simulink model "PvarrayParrallel"  (R2025a)
settings: Solver=ode23tb  StartTime=0.0  StopTime=0.2  RelTol=1e-3
libraries: spsDiodeLib x7, spsPVArrayLib x6, spsSeriesRLCBranchLib x6, slpidlib x2, spsPower3phPhasorLib x2, spsThreePhaseVIMeasurementLib x2, spsVoltageMeasurementLib x2, spsCurrentMeasurementLib x1, spsIGBTDiodeLib x1, eeGeneralControl x1, spsPLL3phLib x1, spsPWMGenerator2LevelLib x1
settings Model: Creator=BIT  LastModifiedBy=BIT

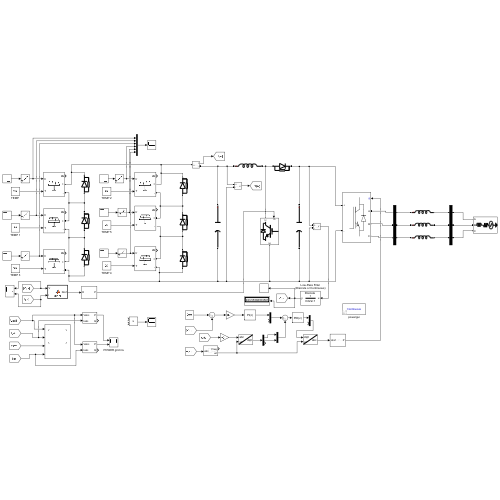
[thumbnail: Simulink's stored preview of the top-level diagram]
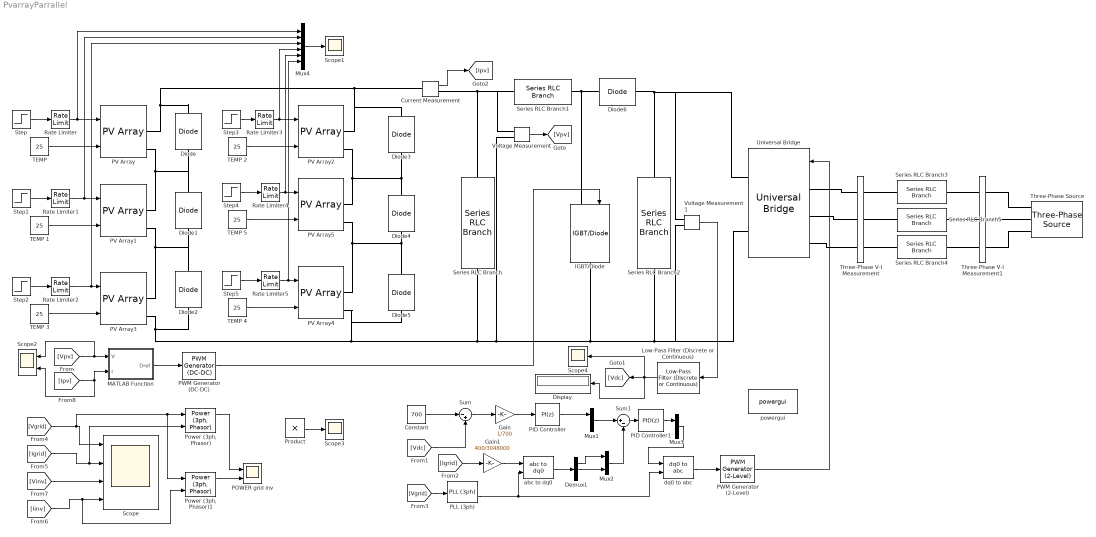
== system PvarrayParrallel ==
  Constant : Constant  Value=700
  Current Measurement : spsCurrentMeasurementLib/Current Measurement  PhasorSimulation=off  OutputType=Complex  PSBequivalent=0
  Demux1 : Demux  Outputs=3
  Diode{,1..6} (7 alike) : spsDiodeLib/Diode  Ron=0.001  Lon=0  Vf=0.8  IC=0  UseSnubber=0  Rs=500  Cs=250e-9  Measurements=off
  Display : Display
  Gain : Gain  Gain=1/700
  Gain1 : Gain  Gain=400/3048000
  IGBT/Diode : spsIGBTDiodeLib/IGBT//Diode  Ron=1e-3  Rs=1e5  Cs=inf  Measurements=off
  Low-Pass Filter (Discrete or Continuous) : eeGeneralControl/Low-Pass Filter (Discrete or Continuous)  K=1  T=1/50  B=inf  A=-inf  init_option=Inherited from block input  x0=0  Ts=1e-06
  MATLAB Function : MATLAB Function  TreatAsAtomicUnit=on
  Mux1 : Mux  Inputs=2
  Mux2 : Mux  Inputs=2
  Mux3 : Mux  Inputs=2
  Mux4 : Mux  Inputs=6
  PID Controller : slpidlib/PID Controller  Controller=PI  Form=Parallel  TimeDomain=Discrete-time  UseExternalTs=off  SampleTime=-1  IntegratorMethod=Forward Euler  FilterMethod=Forward Euler  ControllerParametersSource=internal  P=100  I=100  UseKiTs=off  D=0  UseExternalDerivativeSource=off  N=100  UseFilter=on  TunerSelectOption=Transfer Function Based (PID Tuner App)  InitialConditionSource=internal  InitialConditionForIntegrator=0  InitialConditionForFilter=0  DifferentiatorICPrevScaledInput=0  ExternalReset=none  TrackingMode=off  Kt=1  LimitOutput=off  SatLimitsSource=internal  UpperSaturationLimit=inf  LowerSaturationLimit=-inf  LinearizeAsGain=on  AntiWindupMode=none  Kb=1  LimitIntegrator=off  UpperIntegratorSaturationLimit=inf  LowerIntegratorSaturationLimit=-inf  POutMin=[]  POutMax=[]  IOutMin=[]  IOutMax=[]  DOutMin=[]  DOutMax=[]  NOutMin=[]  NOutMax=[]  SumOutMin=[]  SumOutMax=[]  SaturationOutMin=[]  SaturationOutMax=[]  PParamMin=[]  PParamMax=[]  IParamMin=[]  IParamMax=[]  DParamMin=[]  DParamMax=[]  NParamMin=[]  NParamMax=[]  KbParamMin=[]  KbParamMax=[]  KtParamMin=[]  KtParamMax=[]  KbOutMin=[]  KbOutMax=[]  KtOutMin=[]  KtOutMax=[]  IntegratorOutMin=[]  IntegratorOutMax=[]  FilterOutMin=[]  FilterOutMax=[]  SumI1OutMin=[]  SumI1OutMax=[]  SumI2OutMin=[]  SumI2OutMax=[]  SumI3OutMin=[]  SumI3OutMax=[]  SumI4OutMin=[]  SumI4OutMax=[]  SumDOutMin=[]  SumDOutMax=[]  DifferentiatorOutMin=[]  DifferentiatorOutMax=[]  FilterDiffOutCoefMin=[]  FilterDiffOutCoefMax=[]  ReciprocalOutMin=[]  ReciprocalOutMax=[]  SumDenOutMin=[]  SumDenOutMax=[]  SumNumOutMin=[]  SumNumOutMax=[]  DivideOutMin=[]  DivideOutMax=[]  UdiffTsProdOutMin=[]  UdiffTsProdOutMax=[]  NTsProdOutMin=[]  NTsProdOutMax=[]  UintegralTsProdOutMin=[]  UintegralTsProdOutMax=[]  UngainTsProdOutMin=[]  UngainTsProdOutMax=[]  ClampingZeroOutDataTypeStr=Inherit: Inherit via back propagation  ClampingZeroOutMin=[]  ClampingZeroOutMax=[]  FilterDenConstantOutDataTypeStr=Inherit: Inherit via back propagation  FilterDenConstantOutMin=[]  FilterDenConstantOutMax=[]  PCopyOutDataTypeStr=Inherit: Inherit via back propagation  PCopyOutMin=[]  PCopyOutMax=[]  NCopyOutDataTypeStr=Inherit: Inherit via back propagation  NCopyOutMin=[]  NCopyOutMax=[]  IntegratorContinuousStateAttributes=''  IntegratorStateMustResolveToSignalObject=off  IntegratorRTWStateStorageClass=Auto  FilterContinuousStateAttributes=''  FilterStateMustResolveToSignalObject=off  FilterRTWStateStorageClass=Auto  ParallelPVariant=InternalParameters  IdealPVariant=Disabled  IVariant=InternalParameters  DVariant=Disabled  IntegratorVariant=Discrete  SatVariant=Disabled  AWVariant=Passthrough  PCopyVariant=Disabled  TRVariant=Disabled  FdbkBlocksVariant=Forward  IdealPFdbkVariant=Disabled  SatFdbkVariant=Disabled  DerivativeFilterVariant=Disabled  NVariant=Disabled  NCopyVariant=Disabled_SignalSpec  FilterICVariant=Disabled  IntegratorICVariant=InternalICs  ExternalResetVariant=Disabled  TRSumVariant=Passthrough  SumFdbkVariant=Disabled  SumVariant=Sum_PI  TsampFilterVariant=InternalTs  TsampNgainVariant=Passthrough  TsampIntegralVariant=Disabled_SignalSpec  ExternalSaturationOutDataTypeStr=Inherit: Same as second input  DerivativeSourceVariant=Disabled  PreIntVariant=InternalPreInt
  PID Controller1 : slpidlib/PID Controller  Controller=PID  Form=Parallel  TimeDomain=Discrete-time  UseExternalTs=off  SampleTime=-1  IntegratorMethod=Forward Euler  FilterMethod=Forward Euler  ControllerParametersSource=internal  P=1  I=1  UseKiTs=off  D=0  UseExternalDerivativeSource=off  N=100  UseFilter=on  TunerSelectOption=Transfer Function Based (PID Tuner App)  InitialConditionSource=internal  InitialConditionForIntegrator=0  InitialConditionForFilter=0  DifferentiatorICPrevScaledInput=0  ExternalReset=none  TrackingMode=off  Kt=1  LimitOutput=off  SatLimitsSource=internal  UpperSaturationLimit=inf  LowerSaturationLimit=-inf  LinearizeAsGain=on  AntiWindupMode=none  Kb=1  LimitIntegrator=off  UpperIntegratorSaturationLimit=inf  LowerIntegratorSaturationLimit=-inf  POutMin=[]  POutMax=[]  IOutMin=[]  IOutMax=[]  DOutMin=[]  DOutMax=[]  NOutMin=[]  NOutMax=[]  SumOutMin=[]  SumOutMax=[]  SaturationOutMin=[]  SaturationOutMax=[]  PParamMin=[]  PParamMax=[]  IParamMin=[]  IParamMax=[]  DParamMin=[]  DParamMax=[]  NParamMin=[]  NParamMax=[]  KbParamMin=[]  KbParamMax=[]  KtParamMin=[]  KtParamMax=[]  KbOutMin=[]  KbOutMax=[]  KtOutMin=[]  KtOutMax=[]  IntegratorOutMin=[]  IntegratorOutMax=[]  FilterOutMin=[]  FilterOutMax=[]  SumI1OutMin=[]  SumI1OutMax=[]  SumI2OutMin=[]  SumI2OutMax=[]  SumI3OutMin=[]  SumI3OutMax=[]  SumI4OutMin=[]  SumI4OutMax=[]  SumDOutMin=[]  SumDOutMax=[]  DifferentiatorOutMin=[]  DifferentiatorOutMax=[]  FilterDiffOutCoefMin=[]  FilterDiffOutCoefMax=[]  ReciprocalOutMin=[]  ReciprocalOutMax=[]  SumDenOutMin=[]  SumDenOutMax=[]  SumNumOutMin=[]  SumNumOutMax=[]  DivideOutMin=[]  DivideOutMax=[]  UdiffTsProdOutMin=[]  UdiffTsProdOutMax=[]  NTsProdOutMin=[]  NTsProdOutMax=[]  UintegralTsProdOutMin=[]  UintegralTsProdOutMax=[]  UngainTsProdOutMin=[]  UngainTsProdOutMax=[]  ClampingZeroOutDataTypeStr=Inherit: Inherit via back propagation  ClampingZeroOutMin=[]  ClampingZeroOutMax=[]  FilterDenConstantOutDataTypeStr=Inherit: Inherit via back propagation  FilterDenConstantOutMin=[]  FilterDenConstantOutMax=[]  PCopyOutDataTypeStr=Inherit: Inherit via back propagation  PCopyOutMin=[]  PCopyOutMax=[]  NCopyOutDataTypeStr=Inherit: Inherit via back propagation  NCopyOutMin=[]  NCopyOutMax=[]  IntegratorContinuousStateAttributes=''  IntegratorStateMustResolveToSignalObject=off  IntegratorRTWStateStorageClass=Auto  FilterContinuousStateAttributes=''  FilterStateMustResolveToSignalObject=off  FilterRTWStateStorageClass=Auto  ParallelPVariant=InternalParameters  IdealPVariant=Disabled  IVariant=InternalParameters  DVariant=InternalParameters  IntegratorVariant=Discrete  SatVariant=Disabled  AWVariant=Passthrough  PCopyVariant=Disabled  TRVariant=Disabled  FdbkBlocksVariant=Forward  IdealPFdbkVariant=Disabled  SatFdbkVariant=Disabled  DerivativeFilterVariant=ForwardEulerFilter  NVariant=InternalParameters  NCopyVariant=Disabled  FilterICVariant=InternalICsFilter  IntegratorICVariant=InternalICs  ExternalResetVariant=Disabled  TRSumVariant=Passthrough  SumFdbkVariant=Disabled  SumVariant=Sum_PID  TsampFilterVariant=InternalTs  TsampNgainVariant=Passthrough  TsampIntegralVariant=Disabled_SignalSpec  ExternalSaturationOutDataTypeStr=Inherit: Same as second input  DerivativeSourceVariant=ErrorSignal  PreIntVariant=InternalPreInt
  PLL (3ph) : spsPLL3phLib/PLL (3ph)  Fmin=45  Par_Init=[0, 50]  ParK=[180, 3200, 1]  TcD=1e-4  MaxRateChangeFreq=12  FilterCutOffFreq=25  Ts=0  AGC=on
  POWER grid inv : Scope  NumInputPorts=2
      settings: ActiveDisplayYMinimum=-286453.02616014116  ActiveDisplayYMaximum=399792.88349648647
  PV Array{,1..2,5} (4 alike) : spsPVArrayLib/PV Array  Npar=650  Nser=4  PlotType=array @ 1000 W/m2 & specified temperatures  S_vec="[ 1000  500  100 ]"  Temp_C_vec="[ 45 25  ]"  ModuleName=User-defined  PlotWhenSelected=off  Pm=213.15  Ncell=60  Voc=36.3  Isc=7.84  Vm=29  Im=7.35  beta_Voc_pc=-0.36099  alpha_Isc_pc=0.102  beta_Voc=-0.13104  alpha_Isc=0.0079968  IL=7.8654  I0=2.9273e-10  nI=0.98119  Rsh=313.0553  Rs=0.39381  RobustModel=off  RobustCellTemperature=313.3991  BAL=on  Tc=1e-6  Tfilter=5e-5
  PV Array3 : spsPVArrayLib/PV Array  Npar=650  Nser=3  PlotType=array @ 1000 W/m2 & specified temperatures  S_vec="[ 1000  500  100 ]"  Temp_C_vec="[ 45 25  ]"  ModuleName=User-defined  PlotWhenSelected=off  Pm=213.15  Ncell=60  Voc=36.3  Isc=7.84  Vm=29  Im=7.35  beta_Voc_pc=-0.36099  alpha_Isc_pc=0.102  beta_Voc=-0.13104  alpha_Isc=0.0079968  IL=7.8654  I0=2.9273e-10  nI=0.98119  Rsh=313.0553  Rs=0.39381  RobustModel=off  RobustCellTemperature=313.3991  BAL=on  Tc=1e-6  Tfilter=5e-5
  PV Array4 : spsPVArrayLib/PV Array  Npar=650  Nser=3  PlotType=array @ 1000 W/m2 & specified temperatures  S_vec="[ 1000  500  100 ]"  Temp_C_vec="[ 45 25  ]"  ModuleName=User-defined  PlotWhenSelected=off  Pm=213.15  Ncell=60  Voc=36.3  Isc=7.84  Vm=29  Im=7.35  beta_Voc_pc=-0.36099  alpha_Isc_pc=0.102  beta_Voc=-0.13104  alpha_Isc=0.0079968  IL=7.8654  I0=2.9273e-10  nI=0.98119  Rsh=313.0553  Rs=0.39381  RobustModel=off  RobustCellTemperature=313.3991  BAL=on  Tc=1e-6  Tfilter=5e-5
  PWM Generator (2-Level) : spsPWMGenerator2LevelLib/PWM Generator (2-Level)  ModulatorType=Three-phase bridge (6 pulses)  ModulatorMode=Unsynchronized  Fc=10000  Pc=90  nF=27  MinMax="[ -1  1 ]"  SamplingTechnique=Natural  ModulatingSignals=off  m=0.8  Freq=60  Phase=0  Ts=0  ShowCarrierOutport=off
  PWM Generator (DC-DC) : spsPWMGeneratorDCDCLib/PWM Generator (DC-DC)  Fsw=10000  Ts=0
  "Power (3ph, Phasor)" : spsPower3phPhasorLib/Power (3ph, Phasor)
      settings: LibrarySourceBlock=|
      | sps_lib/Sensors and Measurements/Power
      | (3ph, Phasor)
  "Power (3ph, Phasor)1" : spsPower3phPhasorLib/Power (3ph, Phasor)
      settings: LibrarySourceBlock=|
      | sps_lib/Sensors and Measurements/Power
      | (3ph, Phasor)
  Product : Product
  Rate Limiter{,1..5} (6 alike) : RateLimiter  RisingSlewLimit=10000  FallingSlewLimit=-10000  SampleTimeMode=inherited
  Scope : Scope  NumInputPorts=4
      settings: ActiveDisplayYMinimum=-1597.0632599299197  ActiveDisplayYMaximum=1599.7151178027298
  Scope1 : Scope
      settings: ActiveDisplayYMinimum=900  ActiveDisplayYMaximum=1100  DataLoggingVariableName=ScopeData4
  Scope2 : Scope  NumInputPorts=2
      settings: ActiveDisplayYMinimum=-48.319060451258906  ActiveDisplayYMaximum=434.87154406133027  DataLoggingVariableName=ScopeData2
  Scope3 : Scope
      settings: ActiveDisplayYMinimum=-1  ActiveDisplayYMaximum=1  DataLoggingVariableName=ScopeData3
  Scope4 : Scope
      settings: ActiveDisplayYMinimum=-115.44448544947615  ActiveDisplayYMaximum=1039.0003690452857  DataLoggingVariableName=ScopeData5
  Series RLC Branch : spsSeriesRLCBranchLib/Series RLC Branch  LConnTagsString=__new0  RConnTagsString=__new0  BranchType=C  Resistance=1  Inductance=1e-3  SetiL0=off  InitialCurrent=0  Capacitance=0.0339  Setx0=off  InitialVoltage=0  Measurements=None
  Series RLC Branch1 : spsSeriesRLCBranchLib/Series RLC Branch  LConnTagsString=__new0  RConnTagsString=__new0  BranchType=L  Resistance=1  Inductance=1.8172e-04  SetiL0=off  InitialCurrent=0  Capacitance=0.0339  Setx0=off  InitialVoltage=0  Measurements=None
  Series RLC Branch2 : spsSeriesRLCBranchLib/Series RLC Branch  LConnTagsString=__new0  RConnTagsString=__new0  BranchType=C  Resistance=1  Inductance=1e-3  SetiL0=off  InitialCurrent=0  Capacitance=0.0339  Setx0=off  InitialVoltage=0  Measurements=None
  Series RLC Branch3 : spsSeriesRLCBranchLib/Series RLC Branch  LConnTagsString=__new0  RConnTagsString=__new0  BranchType=L  Resistance=1  Inductance=9.4963e-05  SetiL0=off  InitialCurrent=0  Capacitance=1e-6  Setx0=off  InitialVoltage=0  Measurements=None
  Series RLC Branch4 : spsSeriesRLCBranchLib/Series RLC Branch  LConnTagsString=__new0  RConnTagsString=__new0  BranchType=L  Resistance=1  Inductance=9.4963e-05  SetiL0=off  InitialCurrent=0  Capacitance=1e-6  Setx0=off  InitialVoltage=0  Measurements=None
  Series RLC Branch5 : spsSeriesRLCBranchLib/Series RLC Branch  LConnTagsString=__new0  RConnTagsString=__new0  BranchType=L  Resistance=1  Inductance=9.4963e-05  SetiL0=off  InitialCurrent=0  Capacitance=1e-6  Setx0=off  InitialVoltage=0  Measurements=None
  Step : Step  Before=1000  After=800  SampleTime=0
  Step1 : Step  Before=1000  After=600  SampleTime=0
  Step2 : Step  Before=1000  After=500  SampleTime=0
  Step3 : Step  Before=1000  After=800  SampleTime=0
  Step4 : Step  Before=1000  After=600  SampleTime=0
  Step5 : Step  Before=1000  After=500  SampleTime=0
  Sum : Sum  Inputs=|-+
  Sum1 : Sum  Inputs=|+-
  TEMP {,1..5} (6 alike) : Constant  Value=25
  Three-Phase V-I Measurement : spsThreePhaseVIMeasurementLib/Three-Phase V-I Measurement  VoltageMeasurement=phase-to-phase  SetLabelV=on  LabelV=Vinv  Vpu=off  VpuLL=off  CurrentMeasurement=yes  SetLabelI=on  LabelI=Iinv  Ipu=off  Pbase=100e6  Vbase=500e3  OutputType=Complex  PhasorSimulation=off  PSBequivalent=0
  Three-Phase V-I Measurement1 : spsThreePhaseVIMeasurementLib/Three-Phase V-I Measurement  VoltageMeasurement=phase-to-phase  SetLabelV=on  LabelV=Vgrid  Vpu=off  VpuLL=off  CurrentMeasurement=yes  SetLabelI=on  LabelI=Igrid  Ipu=off  Pbase=100e6  Vbase=500e3  OutputType=Complex  PhasorSimulation=off  PSBequivalent=0
  Three-Phase Source : spsThreePhaseSourceLib/Three-Phase Source  InternalConnection=Yg  VoltagePhases=off  Voltage=400  PhaseAngle=0  Voltage_phases=[25e3 25e3 25e3]/sqrt(3)  PhaseAngles_phases=[0 -120 +120]  Frequency=50  NonIdealSource=on  SpecifyImpedance=off  Resistance=0.8929  Inductance=16.58e-3  ShortCircuitLevel=100e6  BaseVoltage=400  XRratio=7  BusType=swing  Pref=10e3  Qref=0  Prefabc=[10e3, 10e3, 10e3]  Qrefabc=[0, 0, 0]  Qmin=-inf  Qmax=inf
  Universal Bridge : spsUniversalBridgeLib/Universal Bridge  Arms=3  SnubberResistance=1e5  SnubberCapacitance=inf  Device=IGBT / Diodes  Ron=1e-3  Lon=0  ForwardVoltages="[  0  0  ]"  ForwardVoltage=0  GTOparameters=[ 10e-6 , 20e-6 ]  IGBTparameters=[ 1e-6 , 2e-6 ]  Measurements=None  Measurements_2=None  converterType=Rectifier
  Voltage Measurement : spsVoltageMeasurementLib/Voltage Measurement  PhasorSimulation=off  OutputType=Complex  PSBequivalent=0
  Voltage Measurement1 : spsVoltageMeasurementLib/Voltage Measurement  PhasorSimulation=off  OutputType=Complex  PSBequivalent=0
  abc to dq0 : spsabctodq0Lib/abc to dq0  Alignment=90 degrees behind phase A axis
  dq0 to abc : spsdq0toabcLib/dq0 to abc  Alignment=90 degrees behind phase A axis
  powergui : sps_lib/powergui  Priority=1  SimulationMode=Continuous  SampleTime=50e-6  frequency=60  Iterations=50  frequencyindice=50  Pbase=100e6  ErrMax=1e-4  UnitsV=kV  UnitsW=MW  buscounter=0  FunctionMessages=off  echomessages=off  EnableUseOfTLC=off  CurrentSourceSwitches=off  DisableSnubberDevices=off  DisableRonSwitches=off  DisableVfSwitches=off  DisplayEquations=off  AutomaticDiscreteSolvers=off  SolverType=Tustin/Backward Euler (TBE)  Interpol=off  ExternalGateDelay=off  methode=off  Ts=100  x0status=blocks  SPID=on  SwTol=0  HookPort=off  NonlinearTolerance=1e-4  nMaxIteration=100  ContinueOnMaxIteration=off  RestoreLinks=warning  ResistiveCurrentMeasurement=off  Frange=[0:2:500]  Ylog=off  Xlog=on  ShowGrid=off  save=off  variable=ZData  structure=0  ZoomFFT=off  StartTime=0.0  cycles=1  DisplayStyle=1  fundamental=60  FreqAxis=off  MaxFrequency=1000  frequencyindicesteady=1  RmsSteady=1  display=off
  wires:
  "TEMP "/1 -> PV Array/2
  TEMP 1/1 -> PV Array1/2
  TEMP 2/1 -> PV Array2/2
  TEMP 3/1 -> PV Array3/2
  TEMP 4/1 -> PV Array4/2
  TEMP 5/1 -> PV Array5/2
  Voltage Measurement/1 -> [Vpv]
  Voltage Measurement1/1 -> Low-Pass Filter (Discrete or Continuous)/1
  Low-Pass Filter (Discrete or Continuous)/1 -> Scope4/1, Display/1, [Vdc]
  MATLAB Function/1(Dref) -> PWM Generator (DC-DC)/1
  PWM Generator (DC-DC)/1 -> IGBT/Diode/1
  Constant/1 -> Sum/1
  [Vdc] -> Sum/2
  Sum/1 -> Gain/1
  Gain/1 -> PID Controller/1
  PID Controller/1 -> Mux1/1
  Mux1/1 -> Sum1/1
  [Igrid] -> Gain1/1
  Gain1/1 -> abc to dq0/1
  abc to dq0/1 -> Demux1/1
  Demux1/1 -> Mux2/1
  Demux1/2 -> Mux2/2
  Mux2/1 -> Sum1/2
  [Vgrid] -> PLL (3ph)/1
  PLL (3ph)/2 -> abc to dq0/2, dq0 to abc/2
  Sum1/1 -> PID Controller1/1
  Mux3/1 -> dq0 to abc/1
  PID Controller1/1 -> Mux3/1
  dq0 to abc/1 -> PWM Generator (2-Level)/1
  PWM Generator (2-Level)/1 -> Universal Bridge/1
  [Vgrid] -> "Power (3ph, Phasor)1"/1, "Power (3ph, Phasor)"/1, Scope/1
  [Igrid] -> "Power (3ph, Phasor)"/2, Scope/2
  [Vinv] -> Scope/3
  [Iinv] -> "Power (3ph, Phasor)1"/2, Scope/4
  "Power (3ph, Phasor)"/1 -> POWER grid inv/1
  "Power (3ph, Phasor)1"/1 -> POWER grid inv/2
  Product/1 -> Scope3/1
  Step/1 -> Rate Limiter/1
  Rate Limiter/1 -> PV Array/1, Mux4/1
  Step1/1 -> Rate Limiter1/1
  Rate Limiter1/1 -> PV Array1/1, Mux4/2
  Step2/1 -> Rate Limiter2/1
  Rate Limiter2/1 -> Mux4/3, PV Array3/1
  Step3/1 -> Rate Limiter3/1
  Rate Limiter3/1 -> PV Array2/1, Mux4/4
  Step4/1 -> Rate Limiter4/1
  Rate Limiter4/1 -> Mux4/5, PV Array5/1
  Step5/1 -> Rate Limiter5/1
  Rate Limiter5/1 -> Mux4/6, PV Array4/1
  Mux4/1 -> Scope1/1
  Current Measurement/1 -> [Ipv]
  [Vpv] -> Scope2/1, MATLAB Function/1(V)
  [Ipv] -> Scope2/2, MATLAB Function/2(I)
  connections:
  PV Array/RConn1 -- Diode/RConn1 -- Current Measurement/LConn1 -- Diode3/RConn1 -- PV Array2/RConn1
  PV Array/RConn2 -- PV Array1/RConn1 -- Diode1/RConn1 -- Diode/LConn1
  PV Array3/RConn1 -- PV Array1/RConn2 -- Diode1/LConn1 -- Diode2/RConn1
  Diode4/RConn1 -- PV Array5/RConn1 -- PV Array2/RConn2 -- Diode3/LConn1
  Diode5/RConn1 -- PV Array4/RConn1 -- PV Array5/RConn2 -- Diode4/LConn1
  Current Measurement/RConn1 -- Series RLC Branch1/LConn1 -- Voltage Measurement/LConn1 -- Series RLC Branch/LConn1
  Series RLC Branch/RConn1 -- PV Array4/RConn2 -- Diode5/LConn1 -- Diode2/LConn1 -- PV Array3/RConn2 -- Voltage Measurement1/LConn2 -- Universal Bridge/RConn2 -- Series RLC Branch2/RConn1 -- IGBT/Diode/RConn1 -- Voltage Measurement/LConn2
  Series RLC Branch1/RConn1 -- Diode6/LConn1 -- IGBT/Diode/LConn1
  Diode6/RConn1 -- Voltage Measurement1/LConn1 -- Universal Bridge/RConn1 -- Series RLC Branch2/LConn1
  Universal Bridge/LConn1 -- Three-Phase V-I Measurement/LConn1
  Universal Bridge/LConn2 -- Three-Phase V-I Measurement/LConn2
  Universal Bridge/LConn3 -- Three-Phase V-I Measurement/LConn3
  Series RLC Branch3/LConn1 -- Three-Phase V-I Measurement/RConn1
  Series RLC Branch5/LConn1 -- Three-Phase V-I Measurement/RConn2
  Series RLC Branch4/LConn1 -- Three-Phase V-I Measurement/RConn3
  Series RLC Branch3/RConn1 -- Three-Phase V-I Measurement1/LConn1
  Series RLC Branch5/RConn1 -- Three-Phase V-I Measurement1/LConn2
  Series RLC Branch4/RConn1 -- Three-Phase V-I Measurement1/LConn3
  Three-Phase Source/RConn1 -- Three-Phase V-I Measurement1/RConn1
  Three-Phase Source/RConn2 -- Three-Phase V-I Measurement1/RConn2
  Three-Phase Source/RConn3 -- Three-Phase V-I Measurement1/RConn3

== matlab function PvarrayParrallel/MATLAB Function ==
  settings: updateMethod=DISCRETE
  data: V input; Dref output; I input
function Dref = MPPT(V,I)
Dinit = 0.42;
Dmax = 0.9;
Dmin = 0.1;

delDref = 0.00008;

persistent Vold Pold Drefold

if(isempty(Vold))
    Vold = 0;
    Pold = 0;
    Drefold = Dinit;
end 

P=V*I;
dV = V-Vold;
dP = P-Pold;

if dP > 0
    if dV > 0
        Dref = Drefold - delDref;
    else
        Dref = Drefold + delDref;
    end

elseif dP<0
    if dV>0
        Dref = Drefold + delDref;
    else
        Dref = Drefold - delDref;
    end

else
    Dref = Drefold;
end

if Dref > Dmax || Dref < Dmin
    Dref = Drefold;
end

Drefold = Dref;
Pold = P;
Vold = V;
